simulink model "Aerodynamic_Surface"  (R2024a)
settings: Solver=FixedStepDiscrete  StartTime=0.0  StopTime=8  FixedStep=.001  RelTol=1e-3
settings Model: Creator=zz  LastModifiedBy=zz

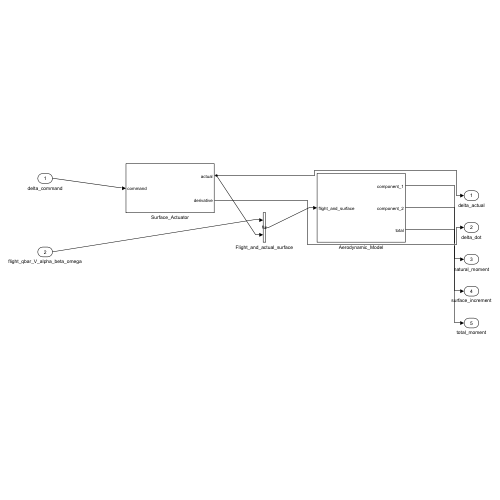
[thumbnail: Simulink's stored preview of the top-level diagram]
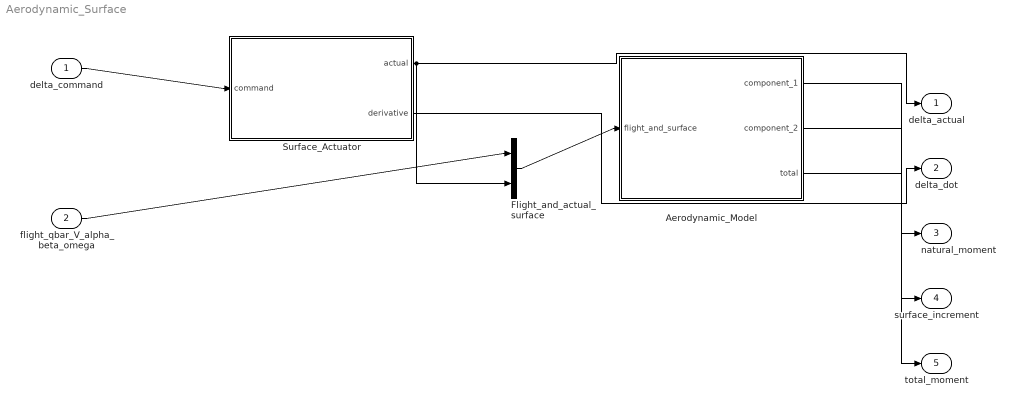
== system Aerodynamic_Surface ==
  delta_command : Inport  PortDimensions=3
  flight_qbar_V_alpha_beta_omega : Inport  Port=2  PortDimensions=7
  Aerodynamic_Model : Subsystem
  Flight_and_actual_surface : Mux  Inputs=2
  Surface_Actuator : Subsystem
  delta_actual : Outport
  delta_dot : Outport  Port=2
  natural_moment : Outport  Port=3
  surface_increment : Outport  Port=4
  total_moment : Outport  Port=5
  wires:
  delta_command/1 -> Surface_Actuator/1(command)
  flight_qbar_V_alpha_beta_omega/1 -> Flight_and_actual_surface/1
  Surface_Actuator/1(actual) -> Flight_and_actual_surface/2, delta_actual/1
  Flight_and_actual_surface/1 -> Aerodynamic_Model/1(flight_and_surface)
  Surface_Actuator/2(derivative) -> delta_dot/1
  Aerodynamic_Model/1(component_1) -> natural_moment/1
  Aerodynamic_Model/2(component_2) -> surface_increment/1
  Aerodynamic_Model/3(total) -> total_moment/1

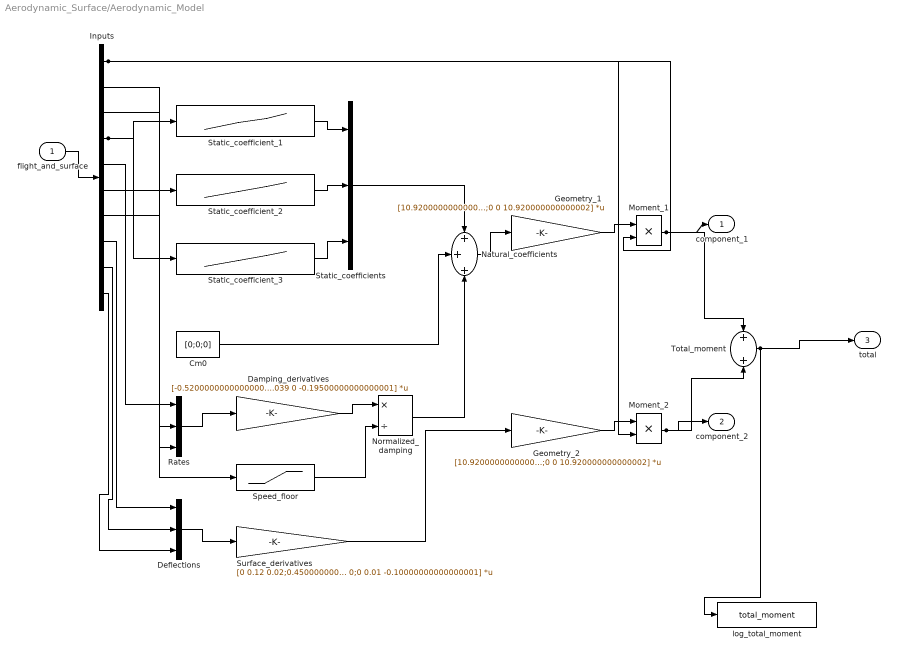
== system Aerodynamic_Surface/Aerodynamic_Model ==
  flight_and_surface : Inport  PortDimensions=10
  Cm0 : Constant  Value=[0;0;0]
  Damping_derivatives : Gain  Gain=[-0.52000000000000002 0 0.13;0 -19.200000000000003 0;-0.039 0 -0.19500000000000001]  Multiplication=Matrix(K*u)
  Deflections : Mux  Inputs=3
  Geometry_1 : Gain  Gain=[10.920000000000002 0 0;0 13.440000000000001 0;0 0 10.920000000000002]  Multiplication=Matrix(K*u)
  Geometry_2 : Gain  Gain=[10.920000000000002 0 0;0 13.440000000000001 0;0 0 10.920000000000002]  Multiplication=Matrix(K*u)
  Inputs : Demux  Outputs=10
  Moment_1 : Product
  Moment_2 : Product
  Natural_coefficients : Sum  Inputs=+++
  Normalized_damping : Product  Inputs=*/
  Rates : Mux  Inputs=3
  Speed_floor : Saturate  UpperLimit=inf  LowerLimit=1
  Static_coefficient_1 : Lookup_n-D  NumberOfTableDimensions=1  BreakpointsForDimension1=[-pi 0 pi]  Table=[0.25132741228718347 0 -0.25132741228718347]
  Static_coefficient_2 : Lookup_n-D  NumberOfTableDimensions=1  BreakpointsForDimension1=[-pi 0 pi]  Table=[1.0995574287564276 0 -1.0995574287564276]
  Static_coefficient_3 : Lookup_n-D  NumberOfTableDimensions=1  BreakpointsForDimension1=[-pi 0 pi]  Table=[-0.37699111843077515 0 0.37699111843077515]
  Static_coefficients : Mux  Inputs=3
  Surface_derivatives : Gain  Gain=[0 0.12 0.02;0.45000000000000001 0 0;0 0.01 -0.10000000000000001]  Multiplication=Matrix(K*u)
  Total_moment : Sum
  log_total_moment : ToWorkspace  VariableName=total_moment  SaveFormat=Timeseries
  component_1 : Outport
  component_2 : Outport  Port=2
  total : Outport  Port=3
  wires:
  flight_and_surface/1 -> Inputs/1
  Inputs/4 -> Static_coefficient_3/1, Static_coefficient_1/1
  Inputs/3 -> Static_coefficient_2/1
  Static_coefficient_1/1 -> Static_coefficients/1
  Static_coefficient_2/1 -> Static_coefficients/2
  Static_coefficient_3/1 -> Static_coefficients/3
  Inputs/5 -> Rates/1
  Inputs/8 -> Deflections/1
  Inputs/6 -> Rates/2
  Inputs/9 -> Deflections/2
  Inputs/7 -> Rates/3
  Inputs/10 -> Deflections/3
  Rates/1 -> Damping_derivatives/1
  Inputs/2 -> Speed_floor/1
  Damping_derivatives/1 -> Normalized_damping/1
  Speed_floor/1 -> Normalized_damping/2
  Deflections/1 -> Surface_derivatives/1
  Static_coefficients/1 -> Natural_coefficients/1
  Cm0/1 -> Natural_coefficients/2
  Normalized_damping/1 -> Natural_coefficients/3
  Natural_coefficients/1 -> Geometry_1/1
  Geometry_1/1 -> Moment_1/1
  Inputs/1 -> Moment_2/2, Moment_1/2
  Moment_1/1 -> Total_moment/1, component_1/1
  Surface_derivatives/1 -> Geometry_2/1
  Geometry_2/1 -> Moment_2/1
  Moment_2/1 -> Total_moment/2, component_2/1
  Total_moment/1 -> log_total_moment/1, total/1

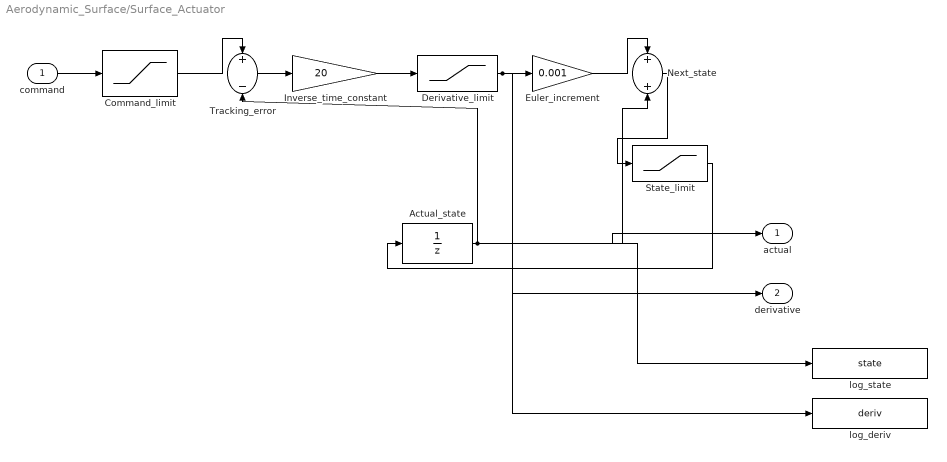
== system Aerodynamic_Surface/Surface_Actuator ==
  command : Inport  PortDimensions=3  SampleTime=0.001
  Actual_state : UnitDelay  InitialCondition=[0;0;0]  SampleTime=0.001
  Command_limit : Saturate  UpperLimit=[0.436332312998582;0.349065850398866;0.349065850398866]  LowerLimit=[-0.436332312998582;-0.349065850398866;-0.349065850398866]
  Derivative_limit : Saturate  UpperLimit=[1.0471975511966;1.0471975511966;1.0471975511966]  LowerLimit=[-1.0471975511966;-1.0471975511966;-1.0471975511966]
  Euler_increment : Gain  Gain=0.001
  Inverse_time_constant : Gain  Gain=20
  Next_state : Sum
  State_limit : Saturate  UpperLimit=[0.436332312998582;0.349065850398866;0.349065850398866]  LowerLimit=[-0.436332312998582;-0.349065850398866;-0.349065850398866]
  Tracking_error : Sum  Inputs=+-
  log_deriv : ToWorkspace  VariableName=deriv  SaveFormat=Timeseries
  log_state : ToWorkspace  VariableName=state  SaveFormat=Timeseries
  actual : Outport
  derivative : Outport  Port=2
  wires:
  command/1 -> Command_limit/1
  Command_limit/1 -> Tracking_error/1
  Actual_state/1 -> log_state/1, actual/1, Next_state/2, Tracking_error/2
  Tracking_error/1 -> Inverse_time_constant/1
  Inverse_time_constant/1 -> Derivative_limit/1
  Derivative_limit/1 -> log_deriv/1, derivative/1, Euler_increment/1
  Euler_increment/1 -> Next_state/1
  Next_state/1 -> State_limit/1
  State_limit/1 -> Actual_state/1
